simulink model "AlKaseeh_PhysicalTwin_PM_FinalScientific_v4_6_2"  (R2025b)
settings: Solver=ode15s  StartTime=0.0  StopTime=9000  MaxStep=0.1  RelTol=1e-4
libraries: fl_lib x34, nesl_utility x24, ee_lib x1, slpidlib x1, SimscapeFluids_lib x1
(part 2 of 2)

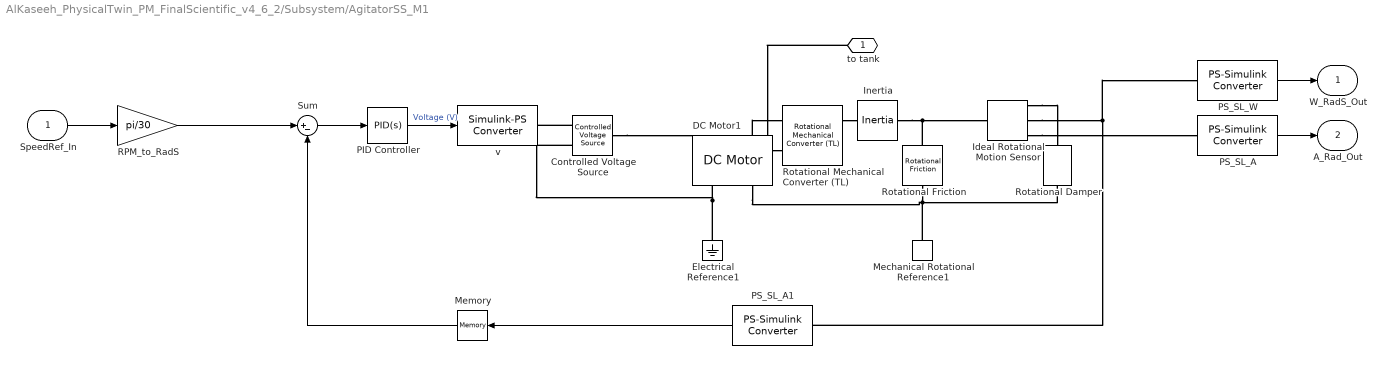
== system AlKaseeh_PhysicalTwin_PM_FinalScientific_v4_6_2/Subsystem/AgitatorSS_M1 ==
  SpeedRef_In : Inport
  Controlled Voltage Source : fl_lib/Electrical/Electrical Sources/Controlled Voltage Source
  DC Motor1 : ee_lib/Electromechanical/Brushed Motors/DC Motor  field_option=ee.enum.field_option.pm  Rf=100 Ohm  Lf=1 H  Laf=0.15 H  If0=0 A  parameterization=ee.enum.dcparam_option.circuit_param  Ra=3.9 Ohm  La=12e-6 H  emf_or_torque=ee.enum.emf_or_torque.kv  Kv=0.072e-3 V/rpm  Ki=6.876e-4 N*m/A  T_stall=0.24e-3 N*m  w_max=19100 rpm  w_rated=15000 rpm  P_rated=0.08 W  V_rated=1.5 V  lam_param=ee.enum.lam_param.damping  i_noload=0 A  V_i_noload=1.5 V  J=0.01 cm^2*g  lam=0 N*m*s/rad  speed0=0 rpm  alpha=3.93e-3 1/K  Tmeas=25 degC  thermal_mass=100 J/K  initial_temperature=25 degC
  Electrical Reference1 : fl_lib/Electrical/Electrical Elements/Electrical Reference
  Ideal Rotational Motion Sensor : fl_lib/Mechanical/Mechanical Sensors/Ideal Rotational Motion Sensor  reference=foundation.enum.MeasurementReference.difference  acceleration_port=false  velocity_port=true  position_port=true  wrap_angle=false  offset=0 rad
  Inertia : fl_lib/Mechanical/Rotational Elements/Inertia  inertia=0.01 kg*m^2  num_ports=foundation.enum.numPorts2.two  w_specify=off  w_priority=High  w=0 rad/s  w_nominal_specify=off  w_nominal_value=1  w_nominal_unit=rad/s  t_specify=off  t_priority=None  t=0 N*m  t_nominal_specify=off  t_nominal_value=1  t_nominal_unit=N*m
      settings: InternalSimscapePortConfiguration="{\"Bottom\":[],\"Left\":[{\"id\":\"I\",\"label\":\"\",\"type\":\"foundation.mechanical.rotational.rotational\"}],\"Right\":[{\"id\":\"J\",\"label\":\"\",\"type\":\"foundation.mechanical.rotational.rotational\"}],\"Top\":[]}"
  Mechanical Rotational Reference1 : fl_lib/Mechanical/Rotational Elements/Mechanical Rotational Reference
  Memory : Memory
  PID Controller : slpidlib/PID Controller  Controller=PID  Form=Parallel  TimeDomain=Continuous-time  UseExternalTs=off  SampleTime=-1  IntegratorMethod=Forward Euler  FilterMethod=Forward Euler  ControllerParametersSource=internal  P=1  I=0.1  UseKiTs=off  D=0  UseExternalDerivativeSource=off  N=100  UseFilter=on  TunerSelectOption=Transfer Function Based (PID Tuner App)  InitialConditionSource=internal  InitialConditionForIntegrator=0  InitialConditionForFilter=0  DifferentiatorICPrevScaledInput=0  ExternalReset=none  TrackingMode=off  Kt=1  LimitOutput=on  SatLimitsSource=internal  UpperSaturationLimit=inf  LowerSaturationLimit=-inf  LinearizeAsGain=on  AntiWindupMode=none  Kb=1  LimitIntegrator=off  UpperIntegratorSaturationLimit=inf  LowerIntegratorSaturationLimit=-inf  POutMin=[]  POutMax=[]  IOutMin=[]  IOutMax=[]  DOutMin=[]  DOutMax=[]  NOutMin=[]  NOutMax=[]  SumOutMin=[]  SumOutMax=[]  SaturationOutMin=[]  SaturationOutMax=[]  PParamMin=[]  PParamMax=[]  IParamMin=[]  IParamMax=[]  DParamMin=[]  DParamMax=[]  NParamMin=[]  NParamMax=[]  KbParamMin=[]  KbParamMax=[]  KtParamMin=[]  KtParamMax=[]  KbOutMin=[]  KbOutMax=[]  KtOutMin=[]  KtOutMax=[]  IntegratorOutMin=[]  IntegratorOutMax=[]  FilterOutMin=[]  FilterOutMax=[]  SumI1OutMin=[]  SumI1OutMax=[]  SumI2OutMin=[]  SumI2OutMax=[]  SumI3OutMin=[]  SumI3OutMax=[]  SumI4OutMin=[]  SumI4OutMax=[]  SumDOutMin=[]  SumDOutMax=[]  DifferentiatorOutMin=[]  DifferentiatorOutMax=[]  FilterDiffOutCoefMin=[]  FilterDiffOutCoefMax=[]  ReciprocalOutMin=[]  ReciprocalOutMax=[]  SumDenOutMin=[]  SumDenOutMax=[]  SumNumOutMin=[]  SumNumOutMax=[]  DivideOutMin=[]  DivideOutMax=[]  UdiffTsProdOutMin=[]  UdiffTsProdOutMax=[]  NTsProdOutMin=[]  NTsProdOutMax=[]  UintegralTsProdOutMin=[]  UintegralTsProdOutMax=[]  UngainTsProdOutMin=[]  UngainTsProdOutMax=[]  ClampingZeroOutDataTypeStr=Inherit: Inherit via back propagation  ClampingZeroOutMin=[]  ClampingZeroOutMax=[]  FilterDenConstantOutDataTypeStr=Inherit: Inherit via back propagation  FilterDenConstantOutMin=[]  FilterDenConstantOutMax=[]  PCopyOutDataTypeStr=Inherit: Inherit via back propagation  PCopyOutMin=[]  PCopyOutMax=[]  NCopyOutDataTypeStr=Inherit: Inherit via back propagation  NCopyOutMin=[]  NCopyOutMax=[]  IntegratorContinuousStateAttributes=''  IntegratorStateMustResolveToSignalObject=off  IntegratorRTWStateStorageClass=Auto  FilterContinuousStateAttributes=''  FilterStateMustResolveToSignalObject=off  FilterRTWStateStorageClass=Auto  ParallelPVariant=InternalParameters  IdealPVariant=Disabled  IVariant=InternalParameters  DVariant=InternalParameters  IntegratorVariant=Continuous  SatVariant=Enabled  AWVariant=Passthrough  PCopyVariant=Disabled  TRVariant=Disabled  FdbkBlocksVariant=Forward  IdealPFdbkVariant=Disabled  SatFdbkVariant=Disabled  DerivativeFilterVariant=ContFilter  NVariant=InternalParameters  NCopyVariant=Disabled  FilterICVariant=InternalICsFilter  IntegratorICVariant=InternalICs  ExternalResetVariant=Disabled  TRSumVariant=Passthrough  SumFdbkVariant=Disabled  SumVariant=Sum_PID  TsampFilterVariant=InternalTs  TsampNgainVariant=Passthrough  TsampIntegralVariant=Disabled_SignalSpec  ExternalSaturationOutDataTypeStr=Inherit: Same as second input  DerivativeSourceVariant=ErrorSignal  PreIntVariant=InternalPreInt
  PS_SL_A : nesl_utility/PS-Simulink Converter  PhysicalDomain=network_engine_domain  SubClassName=ps_output  LeftPortType=input  RightPortType=output  PseudoPeriodic=off  Frequencies=[]  VectorFormat=inherit  Unit=inherit  AffineConversion=off
  PS_SL_A1 : nesl_utility/PS-Simulink Converter  PhysicalDomain=network_engine_domain  SubClassName=ps_output  LeftPortType=input  RightPortType=output  PseudoPeriodic=off  Frequencies=[]  VectorFormat=inherit  Unit=inherit  AffineConversion=off
  PS_SL_W : nesl_utility/PS-Simulink Converter  PhysicalDomain=network_engine_domain  SubClassName=ps_output  LeftPortType=input  RightPortType=output  PseudoPeriodic=off  Frequencies=[]  VectorFormat=inherit  Unit=rad/s  AffineConversion=off
  RPM_to_RadS : Gain  Gain=pi/30
  Rotational Mechanical Converter (TL) : fl_lib/Thermal Liquid/Elements/Rotational Mechanical Converter (TL)  mech_orientation=foundation.enum.MechOrientationRotational.Positive  rotation_spec=foundation.enum.RotationSpec.Calculate  theta0=0 rad  volume_displacement=1e-4 m^3/rad  dead_volume=1e-5 m^3  area=0.01 m^2  environment_spec=foundation.enum.pressure_spec.atmospheric  environment_pressure=0.101325 MPa  dynamic_compressibility=true  p0=0.101325 MPa  T0=293.15 K  p_nominal=0.101325 MPa  T_nominal=293.15 K
      settings: InternalSimscapePortConfiguration="{\"Bottom\":[],\"Left\":[{\"id\":\"A\",\"label\":\"A\",\"type\":\"foundation.thermal_liquid.thermal_liquid\"},{\"id\":\"R\",\"label\":\"R\",\"type\":\"foundation.mechanical.rotational.rotational\"}],\"Right\":[{\"id\":\"H\",\"label\":\"H\",\"type\":\"foundation.thermal.thermal\"},{\"id\":\"C\",\"label\":\"C\",\"type\":\"foundation.mechanical.rotational.rotational\"}],\"Top\":[]}"
  Rotational Damper : fl_lib/Mechanical/Rotational Elements/Rotational Damper  D=0.001 N*m*s/rad  w_specify=off  w_priority=None  w=0 rad/s  w_nominal_specify=off  w_nominal_value=1  w_nominal_unit=rad/s  t_specify=off  t_priority=None  t=0 N*m  t_nominal_specify=on  t_nominal_value=1  t_nominal_unit=N*m
  Rotational Friction : fl_lib/Mechanical/Rotational Elements/Rotational Friction  brkwy_trq=0.5 N*m  brkwy_vel=0.1 rad/s  Col_trq=0.3 N*m  visc_coef=0.02 N*m*s/rad  w_specify=off  w_priority=None  w=0 rad/s  w_nominal_specify=off  w_nominal_value=1  w_nominal_unit=rad/s  t_specify=off  t_priority=None  t=0 N*m  t_nominal_specify=off  t_nominal_value=1  t_nominal_unit=N*m
  Sum : Sum  Inputs=|+-
  v : nesl_utility/Simulink-PS Converter  PhysicalDomain=network_engine_domain  SubClassName=ps_input  LeftPortType=input  RightPortType=output  PseudoPeriodic=off  Frequencies=[]  NoiseDistribution=none  NoiseParameters=[]  Unit=1  AffineConversion=off  FilteringAndDerivatives=provide  SimscapeFilterOrder=1  InputFilterTimeConstant=0.001  UdotUserProvided=0
  to tank : PMIOPort  Side=Left
  W_RadS_Out : Outport
  A_Rad_Out : Outport  Port=2
  wires:
  SpeedRef_In/1 -> RPM_to_RadS/1
  PS_SL_W/1 -> W_RadS_Out/1
  PS_SL_A/1 -> A_Rad_Out/1
  PID Controller/1 -> v/1  "Voltage (V)"
  RPM_to_RadS/1 -> Sum/1
  Sum/1 -> PID Controller/1
  PS_SL_A1/1 -> Memory/1
  Memory/1 -> Sum/2
  connections:
  Electrical Reference1/LConn1 -- Controlled Voltage Source/RConn2 -- DC Motor1/RConn1
  Ideal Rotational Motion Sensor/RConn2 -- PS_SL_A1/LConn1 -- PS_SL_W/LConn1
  Ideal Rotational Motion Sensor/RConn3 -- PS_SL_A/LConn1
  Controlled Voltage Source/RConn1 -- v/RConn1
  Controlled Voltage Source/LConn1 -- DC Motor1/LConn1
  DC Motor1/RConn2 -- Rotational Friction/RConn1 -- Mechanical Rotational Reference1/LConn1 -- Rotational Damper/RConn1
  to tank/RConn1 -- Rotational Mechanical Converter (TL)/LConn1
  DC Motor1/LConn2 -- Rotational Mechanical Converter (TL)/LConn2
  Rotational Mechanical Converter (TL)/RConn2 -- Inertia/LConn1
  Ideal Rotational Motion Sensor/RConn1 -- Rotational Damper/LConn1
  Inertia/RConn1 -- Rotational Friction/LConn1 -- Ideal Rotational Motion Sensor/LConn1

== matlab function AlKaseeh_PhysicalTwin_PM_FinalScientific_v4_6_2/Fault_Injector ==
  settings: updateMethod=DISCRETE  sampleTime=0.1
  data: Prod_InletValve input; Prod_InletValveOut output; Prod_ToTankValve input; Prod_ToFillingValve input; CIP_InletValve input; CIP_ReturnValve input; SteamValve input; CIP_ReturnFlowCmd input; Prod_FillFlowCmd input; AgitatorRPM input; Mode input; CIP_SupplyFlowCmd input; Prod_DischargeFlowCmd input; t input; FaultCode input; FaultSeverity input; FaultStart input; FaultEnd input; Prod_ToTankValveOut output; Prod_ToFillingValveOut output; CIP_InletValveOut output; CIP_ReturnValveOut output; SteamValveOut output; CIP_ReturnFlowCmdOut output; Prod_FillFlowCmdOut output; AgitatorRPMOut output; ModeOut output; CIP_SupplyFlowCmdOut output; Prod_DischargeFlowCmdOut output; FaultActive output; FaultCodeOut output; FaultSeverityOut output
function [Prod_InletValveOut, Prod_ToTankValveOut, Prod_ToFillingValveOut, ...
          CIP_InletValveOut, CIP_ReturnValveOut, SteamValveOut, ...
          CIP_ReturnFlowCmdOut, Prod_FillFlowCmdOut, AgitatorRPMOut, ModeOut, ...
          CIP_SupplyFlowCmdOut, Prod_DischargeFlowCmdOut, ...
          FaultActive, FaultCodeOut, FaultSeverityOut] = ...
          Fault_Injector(Prod_InletValve, Prod_ToTankValve, Prod_ToFillingValve, ...
          CIP_InletValve, CIP_ReturnValve, SteamValve, ...
          CIP_ReturnFlowCmd, Prod_FillFlowCmd, AgitatorRPM, Mode, ...
          CIP_SupplyFlowCmd, Prod_DischargeFlowCmd, ...
          t, FaultCode, FaultSeverity, FaultStart, FaultEnd)
%#codegen
% Al Kaseeh fault injector - Final Scientific v4
%
% Physical fault codes:
%  0 Normal
%  1 Production fill-pump degradation
%  2 CIP supply-pump degradation
%  3 Production inlet-valve blockage
%  4 Tank inlet-valve blockage
%  5 Product discharge-valve blockage
%  6 Product discharge-valve leakage / stuck open
%  7 Heating / steam degradation
%  8 Agitator degradation
%  9 CIP inlet-valve blockage
% 10 CIP return-valve blockage
% 11 Product discharge-pump degradation
% 12 CIP return-pump degradation
%
% Sensor-fault codes 101..106 remain injected in the data-export layer.
%
% Important scientific change:
% FaultActive indicates an EFFECTIVE physical fault, not merely that the
% requested time interval is active. For degradations/blockages, the
% affected component must also be commanded/operating.

VALVE_CLOSE = 1.0e-8;
VALVE_OPEN  = 5.0e-3;

%% Default outputs = unmodified controller commands
Prod_InletValveOut      = Prod_InletValve;
Prod_ToTankValveOut     = Prod_ToTankValve;
Prod_ToFillingValveOut  = Prod_ToFillingValve;
CIP_InletValveOut       = CIP_InletValve;
CIP_ReturnValveOut      = CIP_ReturnValve;
SteamValveOut           = SteamValve;

CIP_ReturnFlowCmdOut     = CIP_ReturnFlowCmd;
Prod_FillFlowCmdOut      = Prod_FillFlowCmd;
CIP_SupplyFlowCmdOut     = CIP_SupplyFlowCmd;
Prod_DischargeFlowCmdOut = Prod_DischargeFlowCmd;

AgitatorRPMOut = AgitatorRPM;
ModeOut = Mode;

severity = min(max(FaultSeverity,0.0),1.0);
requested = (FaultCode > 0.0) && (t >= FaultStart) && (t <= FaultEnd);
effective = false;

if requested
    code = int32(FaultCode);

    switch code

        case int32(1)
            % Production fill pump degradation.
            if Prod_FillFlowCmd > 1.0e-6
                Prod_FillFlowCmdOut = Prod_FillFlowCmd*(1.0-severity);
                effective = true;
            end

        case int32(2)
            % CIP supply pump degradation.
            if CIP_SupplyFlowCmd > 1.0e-6
                CIP_SupplyFlowCmdOut = CIP_SupplyFlowCmd*(1.0-severity);
                effective = true;
            end

        case int32(3)
            % Production inlet valve blockage.
            if Prod_InletValve > (10.0*VALVE_CLOSE)
                Prod_InletValveOut = max(VALVE_CLOSE, ...
                    Prod_InletValve*(1.0-severity));
                effective = true;
            end

        case int32(4)
            % Tank inlet valve blockage.
            if Prod_ToTankValve > (10.0*VALVE_CLOSE)
                Prod_ToTankValveOut = max(VALVE_CLOSE, ...
                    Prod_ToTankValve*(1.0-severity));
                effective = true;
            end

        case int32(5)
            % Product discharge valve blockage.
            if Prod_ToFillingValve > (10.0*VALVE_CLOSE)
                Prod_ToFillingValveOut = max(VALVE_CLOSE, ...
                    Prod_ToFillingValve*(1.0-severity));
                effective = true;
            end

        case int32(6)
            % Product discharge valve leakage/stuck open.
            % Leakage can be physically effective even while the controller
            % requests the valve to be closed.
            forcedOpening = max(VALVE_CLOSE, severity*VALVE_OPEN);
            Prod_ToFillingValveOut = max(Prod_ToFillingValve, forcedOpening);
            effective = true;

        case int32(7)
            % Heating degradation.
            if SteamValve > 1.0e-6
                SteamValveOut = SteamValve*(1.0-severity);
                effective = true;
            end

        case int32(8)
            % Agitator degradation.
            if AgitatorRPM > 1.0e-6
                AgitatorRPMOut = AgitatorRPM*(1.0-severity);
                effective = true;
            end

        case int32(9)
            % CIP inlet valve blockage.
            if CIP_InletValve > (10.0*VALVE_CLOSE)
                CIP_InletValveOut = max(VALVE_CLOSE, ...
                    CIP_InletValve*(1.0-severity));
                effective = true;
            end

        case int32(10)
            % CIP return valve blockage.
            if CIP_ReturnValve > (10.0*VALVE_CLOSE)
                CIP_ReturnValveOut = max(VALVE_CLOSE, ...
                    CIP_ReturnValve*(1.0-severity));
                effective = true;
            end

        case int32(11)
            % Product discharge pump degradation.
            if Prod_DischargeFlowCmd > 1.0e-6
                Prod_DischargeFlowCmdOut = ...
                    Prod_DischargeFlowCmd*(1.0-severity);
                effective = true;
            end

        case int32(12)
            % CIP return pump degradation.
            if CIP_ReturnFlowCmd > 1.0e-6
                CIP_ReturnFlowCmdOut = CIP_ReturnFlowCmd*(1.0-severity);
                effective = true;
            end
    end
end

FaultActive = double(effective);
FaultCodeOut = FaultCode;
FaultSeverityOut = severity;
end

== matlab function AlKaseeh_PhysicalTwin_PM_FinalScientific_v4_6_2/Jameed_Process_Controller ==
  settings: updateMethod=DISCRETE  sampleTime=0.1
  data: t input; Prod_InletValve output; TK1_Level input; TK1_Temp input; Prod_ToTankValve output; Prod_ToFillingValve output; CIP_InletValve output; CIP_ReturnValve output; SteamValve output; CIP_ReturnFlowCmd output; Prod_FillFlowCmd output; AgitatorRPM output; Mode output; CIP_SupplyFlowCmd output; Prod_DischargeFlowCmd output
function [Prod_InletValve, Prod_ToTankValve, Prod_ToFillingValve, ...
          CIP_InletValve, CIP_ReturnValve, SteamValve, ...
          CIP_ReturnFlowCmd, Prod_FillFlowCmd, AgitatorRPM, Mode, ...
          CIP_SupplyFlowCmd, Prod_DischargeFlowCmd] = ...
          Process_Controller(t, TK1_Level, TK1_Temp)
%#codegen
% Final Scientific v4.6.2
% Confirmed fix: Prod_ToTankValve is the SHARED tank inlet used by CIP.
% It must stay OPEN in Mode 5 and during Mode 6 supply ramp-down.

persistent state entryTime lastTime steamLatched
persistent productLowSince cipDrainLowSince cipPermitted

if isempty(state), state=uint8(1); end
if isempty(entryTime), entryTime=0.0; end
if isempty(lastTime), lastTime=-1.0; end
if isempty(steamLatched), steamLatched=true; end
if isempty(productLowSince), productLowSince=-1.0; end
if isempty(cipDrainLowSince), cipDrainLowSince=-1.0; end
if isempty(cipPermitted), cipPermitted=false; end

if t < lastTime
    state=uint8(1);
    entryTime=t;
    steamLatched=true;
    productLowSince=-1.0;
    cipDrainLowSince=-1.0;
    cipPermitted=false;
end
lastTime=t;

VALVE_OPEN  = 5.0e-3;
VALVE_CLOSE = 1.0e-8;

L_FILL_TARGET = 1.45;
L_PRODUCT_TARGET = 0.20;
L_CIP_PERMIT = 0.23;
L_CIP_DRAIN_STOP = 0.07;
L_DRY_PROTECT = 0.04;
L_CIP_HIGH = 1.55;

T_SET = 338.15;
T_LOW = 336.15;
T_HIGH = 340.15;
T_HARD_HIGH = 342.00;

RPM_SET = 23.2;

MIN_MIX_TIME = 300.0;
HOLD_TIME = 600.0;
CIP_CIRC_TIME = 900.0;

FILL_TIMEOUT = 1800.0;
HEAT_TIMEOUT = 6000.0;
DISCHARGE_TIMEOUT = 1800.0;
CIP_DRAIN_TIMEOUT = 900.0;

FILL_VALVE_RELEASE = 1.0;
PROD_DISCHARGE_VALVE_LEAD = 5.0;
PROD_DISCHARGE_RAMP = 5.0;
PRODUCT_LOW_CONFIRM_TIME = 10.0;

CIP_VALVE_LEAD = 5.0;
CIP_PUMP_RAMP = 10.0;
CIP_SUPPLY_RAMPDOWN = 10.0;
CIP_DRAIN_CONFIRM_TIME = 10.0;

% Defaults
Prod_InletValve = VALVE_CLOSE;
Prod_ToTankValve = VALVE_CLOSE;
Prod_ToFillingValve = VALVE_CLOSE;
CIP_InletValve = VALVE_CLOSE;
CIP_ReturnValve = VALVE_CLOSE;
SteamValve = 0.0;

CIP_ReturnFlowCmd = 0.0;
Prod_FillFlowCmd = 0.0;
CIP_SupplyFlowCmd = 0.0;
Prod_DischargeFlowCmd = 0.0;

AgitatorRPM = 0.0;
Mode = 0.0;

elapsed = t-entryTime;

switch state

    case uint8(1)   % Filling
        Mode = 1.0;
        Prod_InletValve = VALVE_OPEN;
        Prod_ToTankValve = VALVE_OPEN;
        Prod_FillFlowCmd = 1.0;

        if TK1_Level >= L_FILL_TARGET
            state=uint8(2);
            entryTime=t;
            steamLatched=true;
        elseif elapsed >= FILL_TIMEOUT
            state=uint8(7);
            entryTime=t;
        end

    case uint8(2)   % Heating + mixing
        Mode = 2.0;
        AgitatorRPM = RPM_SET;

        if elapsed < FILL_VALVE_RELEASE
            Prod_InletValve = VALVE_OPEN;
            Prod_ToTankValve = VALVE_OPEN;
        end

        if TK1_Temp <= T_LOW
            steamLatched=true;
        elseif TK1_Temp >= T_HIGH
            steamLatched=false;
        end

        if steamLatched
            SteamValve=1.0;
        end

        if (TK1_Temp >= T_SET) && (elapsed >= MIN_MIX_TIME)
            state=uint8(3);
            entryTime=t;
        elseif elapsed >= HEAT_TIMEOUT
            state=uint8(7);
            entryTime=t;
        end

    case uint8(3)   % Holding
        Mode = 3.0;
        AgitatorRPM = RPM_SET;

        if TK1_Temp <= T_LOW
            steamLatched=true;
        elseif TK1_Temp >= T_HIGH
            steamLatched=false;
        end

        if steamLatched
            SteamValve=1.0;
        end

        if elapsed >= HOLD_TIME
            state=uint8(4);
            entryTime=t;
            productLowSince=-1.0;
            cipPermitted=false;
        end

    case uint8(4)   % Product discharge
        Mode = 4.0;
        AgitatorRPM = 0.0;
        Prod_ToFillingValve = VALVE_OPEN;

        if elapsed >= PROD_DISCHARGE_VALVE_LEAD
            r=(elapsed-PROD_DISCHARGE_VALVE_LEAD)/PROD_DISCHARGE_RAMP;
            if r < 0.0
                r=0.0;
            elseif r > 1.0
                r=1.0;
            end
            Prod_DischargeFlowCmd=r;
        end

        if TK1_Level <= L_CIP_PERMIT
            Prod_DischargeFlowCmd=0.0;
            if productLowSince < 0.0
                productLowSince=t;
            end
        else
            productLowSince=-1.0;
        end

        if (productLowSince >= 0.0) && ...
                ((t-productLowSince) >= PRODUCT_LOW_CONFIRM_TIME)
            cipPermitted=true;
            state=uint8(5);
            entryTime=t;
            cipDrainLowSince=-1.0;
        elseif elapsed >= DISCHARGE_TIMEOUT
            cipPermitted=false;
            state=uint8(7);
            entryTime=t;
        end

    case uint8(5)   % CIP circulation
        Mode = 5.0;
        AgitatorRPM = 0.0;

        if cipPermitted

            % Isolate production SOURCE.
            Prod_InletValve = VALVE_CLOSE;
            Prod_FillFlowCmd = 0.0;
            Prod_ToFillingValve = VALVE_CLOSE;
            Prod_DischargeFlowCmd = 0.0;

            % v4.6.2 FIX:
            % This is the shared tank inlet and must be OPEN for CIP.
            Prod_ToTankValve = VALVE_OPEN;

            CIP_InletValve = VALVE_OPEN;
            CIP_ReturnValve = VALVE_OPEN;

            if elapsed >= CIP_VALVE_LEAD
                r=(elapsed-CIP_VALVE_LEAD)/CIP_PUMP_RAMP;
                if r < 0.0
                    r=0.0;
                elseif r > 1.0
                    r=1.0;
                end
                CIP_SupplyFlowCmd=r;
                CIP_ReturnFlowCmd=r;
            end

            if TK1_Level >= L_CIP_HIGH
                CIP_SupplyFlowCmd=0.0;
            end

            if TK1_Level <= L_DRY_PROTECT
                CIP_ReturnFlowCmd=0.0;
            end

            if elapsed >= (CIP_VALVE_LEAD + CIP_PUMP_RAMP + CIP_CIRC_TIME)
                state=uint8(6);
                entryTime=t;
                cipDrainLowSince=-1.0;
            end

        else
            state=uint8(7);
            entryTime=t;
        end

    case uint8(6)   % CIP final drain
        Mode = 6.0;
        AgitatorRPM = 0.0;

        if cipPermitted

            % Production source remains isolated.
            Prod_InletValve = VALVE_CLOSE;
            Prod_FillFlowCmd = 0.0;
            Prod_ToFillingValve = VALVE_CLOSE;
            Prod_DischargeFlowCmd = 0.0;

            CIP_ReturnValve = VALVE_OPEN;
            CIP_ReturnFlowCmd = 1.0;

            % v4.6.2 FIX:
            % Keep shared tank inlet open until CIP supply is fully zero.
            if elapsed < CIP_SUPPLY_RAMPDOWN
                Prod_ToTankValve = VALVE_OPEN;
                CIP_InletValve = VALVE_OPEN;

                r=1.0-(elapsed/CIP_SUPPLY_RAMPDOWN);
                if r < 0.0
                    r=0.0;
                elseif r > 1.0
                    r=1.0;
                end
                CIP_SupplyFlowCmd=r;
            else
                CIP_SupplyFlowCmd=0.0;
                CIP_InletValve=VALVE_CLOSE;
                Prod_ToTankValve=VALVE_CLOSE;
            end

            if TK1_Level <= L_CIP_DRAIN_STOP
                CIP_ReturnFlowCmd=0.0;
                if cipDrainLowSince < 0.0
                    cipDrainLowSince=t;
                end
            else
                cipDrainLowSince=-1.0;
            end

            if (cipDrainLowSince >= 0.0) && ...
                    ((t-cipDrainLowSince) >= CIP_DRAIN_CONFIRM_TIME)
                state=uint8(0);
                entryTime=t;
                cipPermitted=false;
            elseif elapsed >= CIP_DRAIN_TIMEOUT
                state=uint8(7);
                entryTime=t;
                cipPermitted=false;
            end

        else
            state=uint8(7);
            entryTime=t;
        end

    case uint8(7)   % Process hold
        Mode = 7.0;
        cipPermitted=false;
        productLowSince=-1.0;
        cipDrainLowSince=-1.0;

    otherwise       % Complete / idle
        Mode = 0.0;
        cipPermitted=false;
end

% Independent safeguards
if TK1_Level <= L_PRODUCT_TARGET
    Prod_DischargeFlowCmd=0.0;
end

if TK1_Temp >= T_HARD_HIGH
    SteamValve=0.0;
end

if TK1_Level <= L_DRY_PROTECT
    AgitatorRPM=0.0;
    SteamValve=0.0;
end

% v4.6.2 corrected CIP interlock:
% isolate production source and filling-line discharge,
% but DO NOT force the shared tank-inlet valve closed.
if (CIP_SupplyFlowCmd > 0.0) || (CIP_ReturnFlowCmd > 0.0)
    Prod_InletValve = VALVE_CLOSE;
    Prod_ToFillingValve = VALVE_CLOSE;
    Prod_FillFlowCmd = 0.0;
    Prod_DischargeFlowCmd = 0.0;
end

if ~cipPermitted
    CIP_InletValve=VALVE_CLOSE;
    CIP_ReturnValve=VALVE_CLOSE;
    CIP_SupplyFlowCmd=0.0;
    CIP_ReturnFlowCmd=0.0;
end

end
